simulink model "rp_spectrometer"  (R2021a)
settings: Solver=FixedStepDiscrete  StartTime=0.0  StopTime=10000  RelTol=1e-3
libraries: xbsIndex_r4 x666, casper_library_misc x8, xps_library x3
(part 1 of 11)
settings Model: Creator=hpw1  LastModifiedBy=mcb
settings SolverCC: AlgebraicLoopSolver=TrustRegion
settings DataIOCC: ReturnWorkspaceOutputs=off
settings OptimizationCC: DefaultParameterBehavior=Inlined
settings DebuggingCC: SFMachineParentedDataDiag=warning  ArithmeticOperatorsInVariantConditions=warning
settings SFSimCC: SimUseLocalCustomCode=off  CustomCodeUndefinedFunction=UseInterfaceOnly
settings RTWCC: RTWUseLocalCustomCode=off

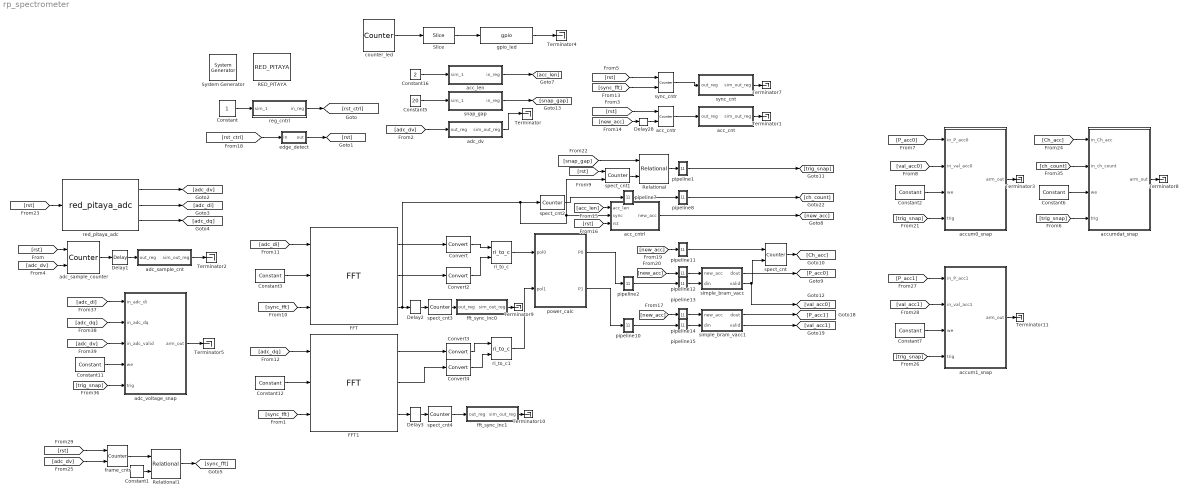
== system rp_spectrometer ==
  " System Generator" : xbsIndex_r4/ System Generator  Tag=genX  xilinxfamily=zynq  part=xc7z010  speed=-1  package=clg400  synthesis_tool=XST  clock_wrapper=Clock Enables  directory=/home/mcb/git/casper/tmp/tutorials_devel/red_pitaya/tut_spec/tut_spec/sysgen  proj_type=Vivado  Synth_file=Vivado Synthesis Defaults  Impl_file=Vivado Implementation Defaults  testbench=off  simulink_period=1  sysclk_period=8  dcm_input_clock_period=10  incr_netlist=off  trim_vbits=Everywhere in SubSystem  dbl_ovrd=According to Block Masks  core_generation=According to Block Masks  run_coregen=off  deprecated_control=off  eval_field=0  block_type=sysgen
  Constant : Constant
  Constant1 : xbsIndex_r4/Constant  const=2^8-1  gui_display_data_type=Fixed-point  arith_type=Unsigned  n_bits=8  bin_pt=0  preci_type=Single  exp_width=8  frac_width=24  explicit_period=off  period=1  equ=P=C  opselect=C  inp2=PCIN>>17  opr=+  inp1=P  carry=CIN  dbl_ovrd=off  block_type=constant
  Constant{2,6..7,11} (4 alike) : xbsIndex_r4/Constant  const=1.0  gui_display_data_type=Boolean  arith_type=Boolean  n_bits=16  bin_pt=14  preci_type=Single  exp_width=8  frac_width=24  explicit_period=on  period=1  equ=P=C  opselect=C  inp2=PCIN>>17  opr=+  inp1=P  carry=CIN  dbl_ovrd=off  block_type=constant
  Constant12 : xbsIndex_r4/Constant  const=0  gui_display_data_type=Fixed-point  arith_type=Signed (2's comp)  n_bits=14  bin_pt=0  preci_type=Single  exp_width=8  frac_width=24  explicit_period=on  period=1  equ=P=C  opselect=C  inp2=PCIN>>17  opr=+  inp1=P  carry=CIN  dbl_ovrd=off  block_type=constant
  Constant16 : Constant  Value=2
  Constant3 : xbsIndex_r4/Constant  const=0  gui_display_data_type=Fixed-point  arith_type=Signed (2's comp)  n_bits=14  bin_pt=0  preci_type=Single  exp_width=8  frac_width=24  explicit_period=on  period=1  equ=P=C  opselect=C  inp2=PCIN>>17  opr=+  inp1=P  carry=CIN  dbl_ovrd=off  block_type=constant
  Constant5 : Constant  Value=20
  Convert{,2..4} (4 alike) : xbsIndex_r4/Convert  gui_display_data_type=Fixed-point  arith_type="Signed  (2's comp)"  n_bits=15  bin_pt=0  float_type=Single  exp_bits=8  fraction_bits=24  quantization=Truncate  overflow=Wrap  en=off  latency=1  pipeline=off  dbl_ovrd=off  block_type=convert
  Delay1 : xbsIndex_r4/Delay  rst=off  infoeditControl=Selection of Reset will increase slice count due to use of real FFs and instead of SRLs  en=off  latency=1  reg_retiming=off  dbl_ovrd=off  block_type=delay
  Delay2 : xbsIndex_r4/Delay  rst=off  infoeditControl=Selection of Reset will increase slice count due to use of real FFs and instead of SRLs  en=off  latency=1  reg_retiming=off  dbl_ovrd=off  block_type=delay
  Delay28 : xbsIndex_r4/Delay  rst=off  infoeditControl=Selection of Reset will increase slice count due to use of real FFs and instead of SRLs  en=off  latency=1  reg_retiming=on  dbl_ovrd=off  block_type=delay
  Delay3 : xbsIndex_r4/Delay  rst=off  infoeditControl=Selection of Reset will increase slice count due to use of real FFs and instead of SRLs  en=off  latency=1  reg_retiming=off  dbl_ovrd=off  block_type=delay
  FFT : xbsIndex_r4/FFT  infoeditControl=Hardware notes: This block implements a burst IO radix-2 architecture if the <b><i>Optimize for</i></b> parameter is selected as <b><i>Resources</i></b>, and the input sample period is 8 times slower than the system sample period; otherwise a pipeline streaming architecture will be used.  transform_length=256  scale_result_by_fft_length=off  bit_reversed_order=on  optimizegoal=Performance  start_frame=on  simulation_type=fast_sim  simulation_model=sysgen:ForwardFFT_Macro  latency=1  block_type=xfft_forward
  FFT1 : xbsIndex_r4/FFT  infoeditControl=Hardware notes: This block implements a burst IO radix-2 architecture if the <b><i>Optimize for</i></b> parameter is selected as <b><i>Resources</i></b>, and the input sample period is 8 times slower than the system sample period; otherwise a pipeline streaming architecture will be used.  transform_length=256  scale_result_by_fft_length=off  bit_reversed_order=on  optimizegoal=Performance  start_frame=on  simulation_type=fast_sim  simulation_model=sysgen:ForwardFFT_Macro  latency=1  block_type=xfft_forward
  RED_PITAYA : xps_library/Platforms/RED_PITAYA  Tag=xps:xsg  hw_sys=RED_PITAYA_14:xc7z010  clk_src=sys_clk  clk_rate=125  sample_period=1  synthesis_tool=XST
      settings: SourceProductName=CASPER XPS Blockset
  Relational : xbsIndex_r4/Relational  mode=a=b  op_type=Bool  en=off  latency=0  dbl_ovrd=off  block_type=relational
  Relational1 : xbsIndex_r4/Relational  mode=a=b  op_type=Bool  en=off  latency=0  dbl_ovrd=off  block_type=relational
  Slice : xbsIndex_r4/Slice  nbits=1  boolean_output=off  mode=Upper Bit Location + Width  bit1=0  base1=MSB of Input  bit0=0  base0=LSB of Input  dbl_ovrd=off  block_type=slice
  Terminator{,1..5,7..11} (11 alike) : Terminator
  acc_cnt : Subsystem  Tag=xps:sw_reg  AncestorBlock=xps_library/Memory/software_register  mask(swreg){io_dir=To Processor, io_delay=0, init_val=0, sample_period=1, names=reg, bitwidths=32, bin_pts=0, arith_types=0, sim_port=on, show_format=off}
      mask prompts: io_dir "I/O direction"; io_delay "I/O delay"; init_val "Initial Value"; sample_period "Sample period"; names "Bitfield names [msb...lsb]"; bitwidths "Bitfield widths"; bin_pts "Bitfield binary pts"; arith_types "Bitfield types, ufix=0, fix=1, bool=2"; sim_port "Provide sim input/output?"; show_format "Print format string?"
      mask help: A 32-bit software-accessible register. Can be divided into bitfields of varying widths and types using the fields in the block mask.
      mask init:
      | swreg_init(gcb)
      settings: AttributesFormatString=1output
      mask TypeOptions io_dir: To Processor | From Processor
      mask Callback io_dir:
      | mask_enables = get_param(gcb, 'MaskEnables');
      | mask_names = get_param(gcb, 'MaskNames');
      | if strcmp(get_param(gcb, 'io_dir'), 'To Processor'),
      |     mask_enables{ismember(mask_names, 'sample_period')} = 'off';
      | else
      |     mask_enables{ismember(mask_names, 'sample_period')} = 'on';
      | end
      | set_param(gcb, 'MaskEnables', mask_enables);
      mask DialogControl ParameterTabVar0 Prompt: Setup
  acc_cntr : xbsIndex_r4/Counter  cnt_type=Free Running  cnt_to=Inf  operation=Up  start_count=0  cnt_by_val=1  arith_type=Unsigned  n_bits=32  bin_pt=0  load_pin=off  rst=on  en=on  explicit_period=on  period=1  use_behavioral_HDL=off  implementation=Fabric  use_rpm=off  dbl_ovrd=off  block_type=counter
  acc_cntrl : Subsystem  mask{chan_bits=8}
      mask prompts: chan_bits "Number of Channels (2^?)"
  acc_len : Subsystem  Tag=xps:sw_reg  AncestorBlock=xps_library/Memory/software_register  mask(swreg){io_dir=From Processor, io_delay=0, init_val=2, sample_period=1, names=reg, bitwidths=32, bin_pts=0, arith_types=0, sim_port=on, show_format=off}
      mask prompts: io_dir "I/O direction"; io_delay "I/O delay"; init_val "Initial Value"; sample_period "Sample period"; names "Bitfield names [msb...lsb]"; bitwidths "Bitfield widths"; bin_pts "Bitfield binary pts"; arith_types "Bitfield types, ufix=0, fix=1, bool=2"; sim_port "Provide sim input/output?"; show_format "Print format string?"
      mask help: A 32-bit software-accessible register. Can be divided into bitfields of varying widths and types using the fields in the block mask.
      mask init:
      | swreg_init(gcb)
      settings: AttributesFormatString=1input
      mask TypeOptions io_dir: To Processor | From Processor
      mask Callback io_dir:
      | mask_enables = get_param(gcb, 'MaskEnables');
      | mask_names = get_param(gcb, 'MaskNames');
      | if strcmp(get_param(gcb, 'io_dir'), 'To Processor'),
      |     mask_enables{ismember(mask_names, 'sample_period')} = 'off';
      | else
      |     mask_enables{ismember(mask_names, 'sample_period')} = 'on';
      | end
      | set_param(gcb, 'MaskEnables', mask_enables);
      mask DialogControl ParameterTabVar0 Prompt: Setup
  accum0_snap : Subsystem  Tag=casper:bitsnap  AncestorBlock=casper_library_scopes/bitfield_snapshot  mask(bitsnap){io_names=[P_acc0 val_acc0], io_widths=[31 1], io_bps=0, io_types=[0 2], show_format=on, snap_storage=bram, snap_dram_dimm=2, snap_dram_clock=250, snap_nsamples=12, snap_data_width=32, snap_offset=off, snap_circap=off, snap_value=off, snap_ext_arm=off, snap_ext_circ=off, snap_provide_outputs=on, snap_use_dsp48=on, snap_delay=0, extra_names=[c d], extra_widths=[30 2], extra_bps=[0 0], extra_types=[0 0]}
      mask prompts: io_names "Names [msb...lsb]"; io_widths "Bitwidths [msb...lsb]"; io_bps "Binary pts [msb...lsb]"; io_types "Data types [msb...lsb], ufix=0, fix=1, bool=2"; show_format "Print format string?"; snap_storage "Storage medium"; snap_dram_dimm "DRAM dimm"; snap_dram_clock "DRAM clock rate"; snap_nsamples "Number of Samples (2^?)"; snap_data_width "Data width"; snap_offset "Start delay support"; snap_circap "Circular capture support"; snap_value "Extra value capture support"; snap_ext_arm "External arm support"; snap_ext_circ "External circular capture support"; snap_provide_outputs "Provide outputs"; snap_use_dsp48 "Use DSP48s to implement counters"; snap_delay "Pre-snapshot delay"; extra_names "Names [msb...lsb]"; extra_widths "Widths [msb...lsb]"; extra_bps "Binary pts [msb...lsb]"; extra_types "Data types [msb...lsb], ufix=0, fix=1, bool=2"
      mask help:
      | A wrapped snapshot block. Allows specification of inputs to a snapblock word so the toolflow can automatically set up the scope.
      | See documentation for snapshot for explanation of parameters.
      mask init:
      | bitsnap_init(gcb);
      settings: AttributesFormatString=|
      | snap(2):uf31.0,b = 32 bits\n32 wide, 4096 deep
      | debugID: 97412755
      mask TypeOptions snap_storage: bram | dram
      mask Callback snap_storage: bitsnap_callback();
      mask TypeOptions snap_dram_dimm: 1 | 2 | 3 | 4
      mask TypeOptions snap_dram_clock: 200 | 250 | 266 | 300 | 333
      mask TypeOptions snap_data_width: 8 | 16 | 32 | 64 | 128
      mask Callback snap_value: bitsnap_callback();
      mask Callback snap_ext_arm: bitsnap_callback();
      mask Callback snap_ext_circ: bitsnap_callback();
      mask Callback snap_provide_outputs: bitsnap_callback();
      mask DialogControl ParameterTabVar0 Prompt: Inputs
      mask DialogControl ParameterTabVar01 Prompt: Snapshot
      mask DialogControl ParameterTabVar012 Prompt: Extra Value
  accum1_snap : Subsystem  Tag=casper:bitsnap  AncestorBlock=casper_library_scopes/bitfield_snapshot  mask(bitsnap){io_names=[P_acc1 val_acc1], io_widths=[31 1], io_bps=0, io_types=[0 2], show_format=on, snap_storage=bram, snap_dram_dimm=2, snap_dram_clock=250, snap_nsamples=12, snap_data_width=32, snap_offset=off, snap_circap=off, snap_value=off, snap_ext_arm=off, snap_ext_circ=off, snap_provide_outputs=on, snap_use_dsp48=on, snap_delay=0, extra_names=[c d], extra_widths=[30 2], extra_bps=[0 0], extra_types=[0 0]}
      mask prompts: io_names "Names [msb...lsb]"; io_widths "Bitwidths [msb...lsb]"; io_bps "Binary pts [msb...lsb]"; io_types "Data types [msb...lsb], ufix=0, fix=1, bool=2"; show_format "Print format string?"; snap_storage "Storage medium"; snap_dram_dimm "DRAM dimm"; snap_dram_clock "DRAM clock rate"; snap_nsamples "Number of Samples (2^?)"; snap_data_width "Data width"; snap_offset "Start delay support"; snap_circap "Circular capture support"; snap_value "Extra value capture support"; snap_ext_arm "External arm support"; snap_ext_circ "External circular capture support"; snap_provide_outputs "Provide outputs"; snap_use_dsp48 "Use DSP48s to implement counters"; snap_delay "Pre-snapshot delay"; extra_names "Names [msb...lsb]"; extra_widths "Widths [msb...lsb]"; extra_bps "Binary pts [msb...lsb]"; extra_types "Data types [msb...lsb], ufix=0, fix=1, bool=2"
      mask help:
      | A wrapped snapshot block. Allows specification of inputs to a snapblock word so the toolflow can automatically set up the scope.
      | See documentation for snapshot for explanation of parameters.
      mask init:
      | bitsnap_init(gcb);
      settings: AttributesFormatString=|
      | snap(2):uf31.0,b = 32 bits\n32 wide, 4096 deep
      | debugID: 34788756
      mask TypeOptions snap_storage: bram | dram
      mask Callback snap_storage: bitsnap_callback();
      mask TypeOptions snap_dram_dimm: 1 | 2 | 3 | 4
      mask TypeOptions snap_dram_clock: 200 | 250 | 266 | 300 | 333
      mask TypeOptions snap_data_width: 8 | 16 | 32 | 64 | 128
      mask Callback snap_value: bitsnap_callback();
      mask Callback snap_ext_arm: bitsnap_callback();
      mask Callback snap_ext_circ: bitsnap_callback();
      mask Callback snap_provide_outputs: bitsnap_callback();
      mask DialogControl ParameterTabVar0 Prompt: Inputs
      mask DialogControl ParameterTabVar01 Prompt: Snapshot
      mask DialogControl ParameterTabVar012 Prompt: Extra Value
  accumdat_snap : Subsystem  Tag=casper:bitsnap  AncestorBlock=casper_library_scopes/bitfield_snapshot  mask(bitsnap){io_names=[Ch_acc ch_count], io_widths=[11 8], io_bps=0, io_types=[0 0], show_format=on, snap_storage=bram, snap_dram_dimm=2, snap_dram_clock=250, snap_nsamples=12, snap_data_width=32, snap_offset=off, snap_circap=off, snap_value=off, snap_ext_arm=off, snap_ext_circ=off, snap_provide_outputs=on, snap_use_dsp48=on, snap_delay=0, extra_names=[c d], extra_widths=[30 2], extra_bps=[0 0], extra_types=[0 0]}
      mask prompts: io_names "Names [msb...lsb]"; io_widths "Bitwidths [msb...lsb]"; io_bps "Binary pts [msb...lsb]"; io_types "Data types [msb...lsb], ufix=0, fix=1, bool=2"; show_format "Print format string?"; snap_storage "Storage medium"; snap_dram_dimm "DRAM dimm"; snap_dram_clock "DRAM clock rate"; snap_nsamples "Number of Samples (2^?)"; snap_data_width "Data width"; snap_offset "Start delay support"; snap_circap "Circular capture support"; snap_value "Extra value capture support"; snap_ext_arm "External arm support"; snap_ext_circ "External circular capture support"; snap_provide_outputs "Provide outputs"; snap_use_dsp48 "Use DSP48s to implement counters"; snap_delay "Pre-snapshot delay"; extra_names "Names [msb...lsb]"; extra_widths "Widths [msb...lsb]"; extra_bps "Binary pts [msb...lsb]"; extra_types "Data types [msb...lsb], ufix=0, fix=1, bool=2"
      mask help:
      | A wrapped snapshot block. Allows specification of inputs to a snapblock word so the toolflow can automatically set up the scope.
      | See documentation for snapshot for explanation of parameters.
      mask init:
      | bitsnap_init(gcb);
      settings: AttributesFormatString=|
      | snap(2):uf11.0,uf8.0 = 19 bits\n32 wide, 4096 deep
      | debugID: 7196602
      mask TypeOptions snap_storage: bram | dram
      mask Callback snap_storage: bitsnap_callback();
      mask TypeOptions snap_dram_dimm: 1 | 2 | 3 | 4
      mask TypeOptions snap_dram_clock: 200 | 250 | 266 | 300 | 333
      mask TypeOptions snap_data_width: 8 | 16 | 32 | 64 | 128
      mask Callback snap_value: bitsnap_callback();
      mask Callback snap_ext_arm: bitsnap_callback();
      mask Callback snap_ext_circ: bitsnap_callback();
      mask Callback snap_provide_outputs: bitsnap_callback();
      mask DialogControl ParameterTabVar0 Prompt: Inputs
      mask DialogControl ParameterTabVar01 Prompt: Snapshot
      mask DialogControl ParameterTabVar012 Prompt: Extra Value
  adc_dv : Subsystem  Tag=xps:sw_reg  AncestorBlock=xps_library/Memory/software_register  mask(swreg){io_dir=To Processor, io_delay=0, init_val=0, sample_period=1, names=reg, bitwidths=1, bin_pts=0, arith_types=2, sim_port=on, show_format=on}
      mask prompts: io_dir "I/O direction"; io_delay "I/O delay"; init_val "Initial Value"; sample_period "Sample period"; names "Bitfield names [msb...lsb]"; bitwidths "Bitfield widths"; bin_pts "Bitfield binary pts"; arith_types "Bitfield types, ufix=0, fix=1, bool=2"; sim_port "Provide sim input/output?"; show_format "Print format string?"
      mask help: A 32-bit software-accessible register. Can be divided into bitfields of varying widths and types using the fields in the block mask.
      mask init:
      | swreg_init(gcb)
      settings: AttributesFormatString=1output:b = 1 bits
      mask TypeOptions io_dir: To Processor | From Processor
      mask Callback io_dir:
      | mask_enables = get_param(gcb, 'MaskEnables');
      | mask_names = get_param(gcb, 'MaskNames');
      | if strcmp(get_param(gcb, 'io_dir'), 'To Processor'),
      |     mask_enables{ismember(mask_names, 'sample_period')} = 'off';
      | else
      |     mask_enables{ismember(mask_names, 'sample_period')} = 'on';
      | end
      | set_param(gcb, 'MaskEnables', mask_enables);
      mask DialogControl ParameterTabVar0 Prompt: Setup
  adc_sample_cnt : Subsystem  Tag=xps:sw_reg  AncestorBlock=xps_library/Memory/software_register  mask(swreg){io_dir=To Processor, io_delay=0, init_val=0, sample_period=1, names=reg, bitwidths=32, bin_pts=0, arith_types=0, sim_port=on, show_format=on}
      mask prompts: io_dir "I/O direction"; io_delay "I/O delay"; init_val "Initial Value"; sample_period "Sample period"; names "Bitfield names [msb...lsb]"; bitwidths "Bitfield widths"; bin_pts "Bitfield binary pts"; arith_types "Bitfield types, ufix=0, fix=1, bool=2"; sim_port "Provide sim input/output?"; show_format "Print format string?"
      mask help: A 32-bit software-accessible register. Can be divided into bitfields of varying widths and types using the fields in the block mask.
      mask init:
      | swreg_init(gcb)
      settings: AttributesFormatString=1output:uf32.0 = 32 bits
      mask TypeOptions io_dir: To Processor | From Processor
      mask Callback io_dir:
      | mask_enables = get_param(gcb, 'MaskEnables');
      | mask_names = get_param(gcb, 'MaskNames');
      | if strcmp(get_param(gcb, 'io_dir'), 'To Processor'),
      |     mask_enables{ismember(mask_names, 'sample_period')} = 'off';
      | else
      |     mask_enables{ismember(mask_names, 'sample_period')} = 'on';
      | end
      | set_param(gcb, 'MaskEnables', mask_enables);
      mask DialogControl ParameterTabVar0 Prompt: Setup
  adc_sample_counter : xbsIndex_r4/Counter  cnt_type=Free Running  cnt_to=Inf  operation=Up  start_count=0  cnt_by_val=1  arith_type=Unsigned  n_bits=32  bin_pt=0  load_pin=off  rst=on  en=on  explicit_period=on  period=1  use_behavioral_HDL=off  implementation=Fabric  dbl_ovrd=off  block_type=counter
  adc_voltage_snap : Subsystem  Tag=casper:bitsnap  AncestorBlock=casper_library_scopes/bitfield_snapshot  mask(bitsnap){io_names=[adc_di adc_dq adc_valid], io_widths=[14 14 1], io_bps=0, io_types=[1 1 2], show_format=on, snap_storage=bram, snap_dram_dimm=2, snap_dram_clock=250, snap_nsamples=12, snap_data_width=32, snap_offset=off, snap_circap=off, snap_value=off, snap_ext_arm=off, snap_ext_circ=off, snap_provide_outputs=on, snap_use_dsp48=on, snap_delay=0, extra_names=[c d], extra_widths=[30 2], extra_bps=[0 0], extra_types=[0 0]}
      mask prompts: io_names "Names [msb...lsb]"; io_widths "Bitwidths [msb...lsb]"; io_bps "Binary pts [msb...lsb]"; io_types "Data types [msb...lsb], ufix=0, fix=1, bool=2"; show_format "Print format string?"; snap_storage "Storage medium"; snap_dram_dimm "DRAM dimm"; snap_dram_clock "DRAM clock rate"; snap_nsamples "Number of Samples (2^?)"; snap_data_width "Data width"; snap_offset "Start delay support"; snap_circap "Circular capture support"; snap_value "Extra value capture support"; snap_ext_arm "External arm support"; snap_ext_circ "External circular capture support"; snap_provide_outputs "Provide outputs"; snap_use_dsp48 "Use DSP48s to implement counters"; snap_delay "Pre-snapshot delay"; extra_names "Names [msb...lsb]"; extra_widths "Widths [msb...lsb]"; extra_bps "Binary pts [msb...lsb]"; extra_types "Data types [msb...lsb], ufix=0, fix=1, bool=2"
      mask help:
      | A wrapped snapshot block. Allows specification of inputs to a snapblock word so the toolflow can automatically set up the scope.
      | See documentation for snapshot for explanation of parameters.
      mask init:
      | bitsnap_init(gcb);
      settings: AttributesFormatString=|
      | snap(3):f14.0,f14.0,b = 29 bits\n32 wide, 4096 deep
      | debugID: 53243759
      mask TypeOptions snap_storage: bram | dram
      mask Callback snap_storage: bitsnap_callback();
      mask TypeOptions snap_dram_dimm: 1 | 2 | 3 | 4
      mask TypeOptions snap_dram_clock: 200 | 250 | 266 | 300 | 333
      mask TypeOptions snap_data_width: 8 | 16 | 32 | 64 | 128
      mask Callback snap_value: bitsnap_callback();
      mask Callback snap_ext_arm: bitsnap_callback();
      mask Callback snap_ext_circ: bitsnap_callback();
      mask Callback snap_provide_outputs: bitsnap_callback();
      mask DialogControl ParameterTabVar0 Prompt: Inputs
      mask DialogControl ParameterTabVar01 Prompt: Snapshot
      mask DialogControl ParameterTabVar012 Prompt: Extra Value
  counter_led : xbsIndex_r4/Counter  cnt_type=Free Running  cnt_to=Inf  operation=Up  start_count=0  cnt_by_val=1  arith_type=Unsigned  n_bits=27  bin_pt=0  load_pin=off  rst=off  en=off  explicit_period=on  period=1  use_behavioral_HDL=off  implementation=Fabric  dbl_ovrd=off  block_type=counter
  edge_detect : Subsystem  AncestorBlock=casper_library_misc/edge_detect  mask(edge_detect){edge=Rising, polarity=Active High, x_in=[0 0.08 0.08 0.16 0.16 0.24 0.24 0.32 0.32 0.4], y_in=[-1 -1  1  1  1  1  1  1  1  1], x_out=[0.6 0.68 0.68 0.76 0.76 0.84 0.84 0.92 0.92 1], y_out=[-1 -1  1  1 -1 -1 -1 -1 -1 -1]}
      mask prompts: edge "Edge Type"; polarity "Output Polarity"; x_in "Input X Positions"; y_in "Input Y Positions"; x_out "Output X Positions"; y_out "Output Y Positions"
      mask help: Output is active for one-cycle after each edge of the specified type (i.e. rising, falling or both).
      mask init:
      | edge_detect_init(gcb,...
      |     'edge',edge,...
      |     'polarity',polarity,...
      |     'x_in',x_in,...
      |     'x_out',x_out,...
      |     'y_in',y_in,...
      |     'y_out',y_out);
      | 
      | x_in_num=str2num(getfield(getfield(get_param(gcb,'UserData'),'parameters'),'x_in'));
      | x_out_num=str2num(getfield(getfield(get_param(gcb,'UserData'),'parameters'),'x_out'));
      | y_in_num=str2num(getfield(getfield(get_param(gcb,'UserData'),'parameters'),'y_in'));
      | y_out_num=str2num(getfield(getfield(get_param(gcb,'UserData'),'parameters'),'y_out'));
      settings: AttributesFormatString=|
      | rising edges
      | active high
      mask Help: Output is active for one-cycle after each edge of the specified type (i.e. rising, falling, or both).  Latency is zero.
      mask TypeOptions edge: Rising | Falling | Both
      mask TypeOptions polarity: Active High | Active Low
      mask Display:
      | plot(x_in_num,0.5+y_in_num*0.2);
      | plot(x_out_num,0.5+y_out_num*0.2);
  fft_sync_inc0 : Subsystem  Tag=xps:sw_reg  AncestorBlock=xps_library/Memory/software_register  mask(swreg){io_dir=To Processor, io_delay=0, init_val=0, sample_period=1, names=reg, bitwidths=8, bin_pts=0, arith_types=0, sim_port=on, show_format=on}
      mask prompts: io_dir "I/O direction"; io_delay "I/O delay"; init_val "Initial Value"; sample_period "Sample period"; names "Bitfield names [msb...lsb]"; bitwidths "Bitfield widths"; bin_pts "Bitfield binary pts"; arith_types "Bitfield types, ufix=0, fix=1, bool=2"; sim_port "Provide sim input/output?"; show_format "Print format string?"
      mask help: A 32-bit software-accessible register. Can be divided into bitfields of varying widths and types using the fields in the block mask.
      mask init:
      | swreg_init(gcb)
      settings: AttributesFormatString=1output:uf8.0 = 8 bits
      mask TypeOptions io_dir: To Processor | From Processor
      mask Callback io_dir:
      | mask_enables = get_param(gcb, 'MaskEnables');
      | mask_names = get_param(gcb, 'MaskNames');
      | if strcmp(get_param(gcb, 'io_dir'), 'To Processor'),
      |     mask_enables{ismember(mask_names, 'sample_period')} = 'off';
      | else
      |     mask_enables{ismember(mask_names, 'sample_period')} = 'on';
      | end
      | set_param(gcb, 'MaskEnables', mask_enables);
      mask DialogControl ParameterTabVar0 Prompt: Setup
  fft_sync_inc1 : Subsystem  Tag=xps:sw_reg  AncestorBlock=xps_library/Memory/software_register  mask(swreg){io_dir=To Processor, io_delay=0, init_val=0, sample_period=1, names=reg, bitwidths=8, bin_pts=0, arith_types=0, sim_port=on, show_format=on}
      mask prompts: io_dir "I/O direction"; io_delay "I/O delay"; init_val "Initial Value"; sample_period "Sample period"; names "Bitfield names [msb...lsb]"; bitwidths "Bitfield widths"; bin_pts "Bitfield binary pts"; arith_types "Bitfield types, ufix=0, fix=1, bool=2"; sim_port "Provide sim input/output?"; show_format "Print format string?"
      mask help: A 32-bit software-accessible register. Can be divided into bitfields of varying widths and types using the fields in the block mask.
      mask init:
      | swreg_init(gcb)
      settings: AttributesFormatString=1output:uf8.0 = 8 bits
      mask TypeOptions io_dir: To Processor | From Processor
      mask Callback io_dir:
      | mask_enables = get_param(gcb, 'MaskEnables');
      | mask_names = get_param(gcb, 'MaskNames');
      | if strcmp(get_param(gcb, 'io_dir'), 'To Processor'),
      |     mask_enables{ismember(mask_names, 'sample_period')} = 'off';
      | else
      |     mask_enables{ismember(mask_names, 'sample_period')} = 'on';
      | end
      | set_param(gcb, 'MaskEnables', mask_enables);
      mask DialogControl ParameterTabVar0 Prompt: Setup
  frame_cntr : xbsIndex_r4/Counter  cnt_type=Free Running  cnt_to=Inf  operation=Up  start_count=0  cnt_by_val=1  arith_type=Unsigned  n_bits=8  bin_pt=0  load_pin=off  rst=on  en=on  explicit_period=on  period=1  use_behavioral_HDL=off  implementation=Fabric  dbl_ovrd=off  block_type=counter
  gpio_led : xps_library/IO/gpio  Tag=xps:gpio  io_group_params_forwarded=on  io_group=ROACH:led  io_group_real=led  io_group_custom=0  io_dir=out  arith_type=Boolean  bitwidth=1  bin_pt=0  bit_index=0  sample_period=1  use_single_ended=off  use_ddr=off  reg_iob=on  reg_clk_phase=0  termination=None  use_iodelay=off
      settings: SourceProductName=CASPER XPS Blockset
  pipeline1 : Subsystem  AncestorBlock=casper_library_delays/pipeline  mask(pipeline){csp_latency=1}
      mask prompts: csp_latency "Latency"
      mask help:
      | An explicitly laid-out delay line to avoid mapping to SRL16s
      | for use in pipelining to help achieve timing closure.
      mask init:
      | pipeline_init(gcb,'latency',csp_latency);
      settings: AttributesFormatString=Latency = %<latency>
      mask Display:
      | port_label('input', 1, 'd');
      | port_label('output', 1, 'q');
      | disp(['Z^-', num2str(csp_latency)]);
  pipeline10 : Subsystem  AncestorBlock=casper_library_delays/pipeline  mask(pipeline){csp_latency=1}
      mask prompts: csp_latency "Latency"
      mask help:
      | An explicitly laid-out delay line to avoid mapping to SRL16s
      | for use in pipelining to help achieve timing closure.
      mask init:
      | pipeline_init(gcb,'latency',csp_latency);
      settings: AttributesFormatString=Latency = %<latency>
      mask Display:
      | port_label('input', 1, 'd');
      | port_label('output', 1, 'q');
      | disp(['Z^-', num2str(csp_latency)]);
  pipeline11 : Subsystem  AncestorBlock=casper_library_delays/pipeline  mask(pipeline){csp_latency=1}
      mask prompts: csp_latency "Latency"
      mask help:
      | An explicitly laid-out delay line to avoid mapping to SRL16s
      | for use in pipelining to help achieve timing closure.
      mask init:
      | pipeline_init(gcb,'latency',csp_latency);
      settings: AttributesFormatString=Latency = %<latency>
      mask Display:
      | port_label('input', 1, 'd');
      | port_label('output', 1, 'q');
      | disp(['Z^-', num2str(csp_latency)]);
  pipeline12 : Subsystem  AncestorBlock=casper_library_delays/pipeline  mask(pipeline){csp_latency=1}
      mask prompts: csp_latency "Latency"
      mask help:
      | An explicitly laid-out delay line to avoid mapping to SRL16s
      | for use in pipelining to help achieve timing closure.
      mask init:
      | pipeline_init(gcb,'latency',csp_latency);
      settings: AttributesFormatString=Latency = %<latency>
      mask Display:
      | port_label('input', 1, 'd');
      | port_label('output', 1, 'q');
      | disp(['Z^-', num2str(csp_latency)]);
  pipeline13 : Subsystem  AncestorBlock=casper_library_delays/pipeline  mask(pipeline){csp_latency=1}
      mask prompts: csp_latency "Latency"
      mask help:
      | An explicitly laid-out delay line to avoid mapping to SRL16s
      | for use in pipelining to help achieve timing closure.
      mask init:
      | pipeline_init(gcb,'latency',csp_latency);
      settings: AttributesFormatString=Latency = %<latency>
      mask Display:
      | port_label('input', 1, 'd');
      | port_label('output', 1, 'q');
      | disp(['Z^-', num2str(csp_latency)]);
  pipeline14 : Subsystem  AncestorBlock=casper_library_delays/pipeline  mask(pipeline){csp_latency=1}
      mask prompts: csp_latency "Latency"
      mask help:
      | An explicitly laid-out delay line to avoid mapping to SRL16s
      | for use in pipelining to help achieve timing closure.
      mask init:
      | pipeline_init(gcb,'latency',csp_latency);
      settings: AttributesFormatString=Latency = %<latency>
      mask Display:
      | port_label('input', 1, 'd');
      | port_label('output', 1, 'q');
      | disp(['Z^-', num2str(csp_latency)]);
  pipeline15 : Subsystem  AncestorBlock=casper_library_delays/pipeline  mask(pipeline){csp_latency=1}
      mask prompts: csp_latency "Latency"
      mask help:
      | An explicitly laid-out delay line to avoid mapping to SRL16s
      | for use in pipelining to help achieve timing closure.
      mask init:
      | pipeline_init(gcb,'latency',csp_latency);
      settings: AttributesFormatString=Latency = %<latency>
      mask Display:
      | port_label('input', 1, 'd');
      | port_label('output', 1, 'q');
      | disp(['Z^-', num2str(csp_latency)]);
  pipeline2 : Subsystem  AncestorBlock=casper_library_delays/pipeline  mask(pipeline){csp_latency=1}
      mask prompts: csp_latency "Latency"
      mask help:
      | An explicitly laid-out delay line to avoid mapping to SRL16s
      | for use in pipelining to help achieve timing closure.
      mask init:
      | pipeline_init(gcb,'latency',csp_latency);
      settings: AttributesFormatString=Latency = %<latency>
      mask Display:
      | port_label('input', 1, 'd');
      | port_label('output', 1, 'q');
      | disp(['Z^-', num2str(csp_latency)]);
  pipeline7 : Subsystem  AncestorBlock=casper_library_delays/pipeline  mask(pipeline){csp_latency=1}
      mask prompts: csp_latency "Latency"
      mask help:
      | An explicitly laid-out delay line to avoid mapping to SRL16s
      | for use in pipelining to help achieve timing closure.
      mask init:
      | pipeline_init(gcb,'latency',csp_latency);
      settings: AttributesFormatString=Latency = %<latency>
      mask Display:
      | port_label('input', 1, 'd');
      | port_label('output', 1, 'q');
      | disp(['Z^-', num2str(csp_latency)]);
  pipeline8 : Subsystem  AncestorBlock=casper_library_delays/pipeline  mask(pipeline){csp_latency=1}
      mask prompts: csp_latency "Latency"
      mask help:
      | An explicitly laid-out delay line to avoid mapping to SRL16s
      | for use in pipelining to help achieve timing closure.
      mask init:
      | pipeline_init(gcb,'latency',csp_latency);
      settings: AttributesFormatString=Latency = %<latency>
      mask Display:
      | port_label('input', 1, 'd');
      | port_label('output', 1, 'q');
      | disp(['Z^-', num2str(csp_latency)]);
  power_calc : Subsystem
  red_pitaya_adc : xps_library/ADCs/red_pitaya_adc  Tag=xps:red_pitaya_adc  bits=14
      settings: SourceProductName=CASPER XPS Blockset
  reg_cntrl : Subsystem  Tag=xps:sw_reg  AncestorBlock=xps_library/Memory/software_register  mask(swreg){io_dir=From Processor, io_delay=0, init_val=0, sample_period=1, names=reg, bitwidths=1, bin_pts=0, arith_types=2, sim_port=on, show_format=on}
      mask prompts: io_dir "I/O direction"; io_delay "I/O delay"; init_val "Initial Value"; sample_period "Sample period"; names "Bitfield names [msb...lsb]"; bitwidths "Bitfield widths"; bin_pts "Bitfield binary pts"; arith_types "Bitfield types, ufix=0, fix=1, bool=2"; sim_port "Provide sim input/output?"; show_format "Print format string?"
      mask help: A 32-bit software-accessible register. Can be divided into bitfields of varying widths and types using the fields in the block mask.
      mask init:
      | swreg_init(gcb)
      settings: AttributesFormatString=1input:b = 1 bits
      mask TypeOptions io_dir: To Processor | From Processor
      mask Callback io_dir:
      | mask_enables = get_param(gcb, 'MaskEnables');
      | mask_names = get_param(gcb, 'MaskNames');
      | if strcmp(get_param(gcb, 'io_dir'), 'To Processor'),
      |     mask_enables{ismember(mask_names, 'sample_period')} = 'off';
      | else
      |     mask_enables{ismember(mask_names, 'sample_period')} = 'on';
      | end
      | set_param(gcb, 'MaskEnables', mask_enables);
      mask DialogControl ParameterTabVar0 Prompt: Setup
  ri_to_c : casper_library_misc/ri_to_c
      settings: SourceProductName=CASPER DSP Blockset
  ri_to_c1 : casper_library_misc/ri_to_c
      settings: SourceProductName=CASPER DSP Blockset
  simple_bram_vacc : Subsystem  AncestorBlock=casper_library_accumulators/simple_bram_vacc  mask(simple_bram_vacc){vec_len=256, arith_type=Unsigned, n_bits=31, bin_pt=0}
      mask prompts: vec_len "Vector length:"; arith_type "Output type:"; n_bits "Bit width (output):"; bin_pt "Binary point (output):"
      mask help: This simple vector accumulator is based on a shift register. It outputs its previous accumulated vector after a new_acc pulse is received.
      mask init:
      | simple_bram_vacc_init(gcb, ...
      |     'vec_len', vec_len, ...
      |     'arith_type', arith_type, ...
      |     'n_bits', n_bits, ...
      |     'bin_pt', bin_pt);
      mask TypeOptions arith_type: Signed | Unsigned
  simple_bram_vacc1 : Subsystem  AncestorBlock=casper_library_accumulators/simple_bram_vacc  mask(simple_bram_vacc){vec_len=256, arith_type=Unsigned, n_bits=31, bin_pt=0}
      mask prompts: vec_len "Vector length:"; arith_type "Output type:"; n_bits "Bit width (output):"; bin_pt "Binary point (output):"
      mask help: This simple vector accumulator is based on a shift register. It outputs its previous accumulated vector after a new_acc pulse is received.
      mask init:
      | simple_bram_vacc_init(gcb, ...
      |     'vec_len', vec_len, ...
      |     'arith_type', arith_type, ...
      |     'n_bits', n_bits, ...
      |     'bin_pt', bin_pt);
      mask TypeOptions arith_type: Signed | Unsigned
  snap_gap : Subsystem  Tag=xps:sw_reg  AncestorBlock=xps_library/Memory/software_register  mask(swreg){io_dir=From Processor, io_delay=0, init_val=20, sample_period=1, names=reg, bitwidths=32, bin_pts=0, arith_types=0, sim_port=on, show_format=off}
      mask prompts: io_dir "I/O direction"; io_delay "I/O delay"; init_val "Initial Value"; sample_period "Sample period"; names "Bitfield names [msb...lsb]"; bitwidths "Bitfield widths"; bin_pts "Bitfield binary pts"; arith_types "Bitfield types, ufix=0, fix=1, bool=2"; sim_port "Provide sim input/output?"; show_format "Print format string?"
      mask help: A 32-bit software-accessible register. Can be divided into bitfields of varying widths and types using the fields in the block mask.
      mask init:
      | swreg_init(gcb)
      settings: AttributesFormatString=1input
      mask TypeOptions io_dir: To Processor | From Processor
      mask Callback io_dir:
      | mask_enables = get_param(gcb, 'MaskEnables');
      | mask_names = get_param(gcb, 'MaskNames');
      | if strcmp(get_param(gcb, 'io_dir'), 'To Processor'),
      |     mask_enables{ismember(mask_names, 'sample_period')} = 'off';
      | else
      |     mask_enables{ismember(mask_names, 'sample_period')} = 'on';
      | end
      | set_param(gcb, 'MaskEnables', mask_enables);
      mask DialogControl ParameterTabVar0 Prompt: Setup
  spect_cnt : xbsIndex_r4/Counter  cnt_type=Free Running  cnt_to=Inf  operation=Up  start_count=0  cnt_by_val=1  arith_type=Unsigned  n_bits=10+1  bin_pt=0  load_pin=off  rst=on  en=on  explicit_period=on  period=1  use_behavioral_HDL=off  implementation=Fabric  use_rpm=off  dbl_ovrd=off  block_type=counter
  spect_cnt1 : xbsIndex_r4/Counter  cnt_type=Free Running  cnt_to=Inf  operation=Up  start_count=0  cnt_by_val=1  arith_type=Unsigned  n_bits=10+1  bin_pt=0  load_pin=off  rst=on  en=on  explicit_period=on  period=1  use_behavioral_HDL=off  implementation=Fabric  use_rpm=off  dbl_ovrd=off  block_type=counter
  spect_cnt2 : xbsIndex_r4/Counter  cnt_type=Free Running  cnt_to=Inf  operation=Up  start_count=0  cnt_by_val=1  arith_type=Unsigned  n_bits=8  bin_pt=0  load_pin=off  rst=on  en=off  explicit_period=on  period=1  use_behavioral_HDL=off  implementation=Fabric  use_rpm=off  dbl_ovrd=off  block_type=counter
  spect_cnt3 : xbsIndex_r4/Counter  cnt_type=Free Running  cnt_to=Inf  operation=Up  start_count=0  cnt_by_val=1  arith_type=Unsigned  n_bits=8  bin_pt=0  load_pin=off  rst=off  en=on  explicit_period=on  period=1  use_behavioral_HDL=off  implementation=Fabric  use_rpm=off  dbl_ovrd=off  block_type=counter
  spect_cnt4 : xbsIndex_r4/Counter  cnt_type=Free Running  cnt_to=Inf  operation=Up  start_count=0  cnt_by_val=1  arith_type=Unsigned  n_bits=8  bin_pt=0  load_pin=off  rst=off  en=on  explicit_period=on  period=1  use_behavioral_HDL=off  implementation=Fabric  use_rpm=off  dbl_ovrd=off  block_type=counter
  sync_cnt : Subsystem  Tag=xps:sw_reg  AncestorBlock=xps_library/Memory/software_register  mask(swreg){io_dir=To Processor, io_delay=0, init_val=0, sample_period=1, names=reg, bitwidths=32, bin_pts=0, arith_types=0, sim_port=on, show_format=off}
      mask prompts: io_dir "I/O direction"; io_delay "I/O delay"; init_val "Initial Value"; sample_period "Sample period"; names "Bitfield names [msb...lsb]"; bitwidths "Bitfield widths"; bin_pts "Bitfield binary pts"; arith_types "Bitfield types, ufix=0, fix=1, bool=2"; sim_port "Provide sim input/output?"; show_format "Print format string?"
      mask help: A 32-bit software-accessible register. Can be divided into bitfields of varying widths and types using the fields in the block mask.
      mask init:
      | swreg_init(gcb)
      settings: AttributesFormatString=1output
      mask TypeOptions io_dir: To Processor | From Processor
      mask Callback io_dir:
      | mask_enables = get_param(gcb, 'MaskEnables');
      | mask_names = get_param(gcb, 'MaskNames');
      | if strcmp(get_param(gcb, 'io_dir'), 'To Processor'),
      |     mask_enables{ismember(mask_names, 'sample_period')} = 'off';
      | else
      |     mask_enables{ismember(mask_names, 'sample_period')} = 'on';
      | end
      | set_param(gcb, 'MaskEnables', mask_enables);
      mask DialogControl ParameterTabVar0 Prompt: Setup
  sync_cntr : xbsIndex_r4/Counter  cnt_type=Free Running  cnt_to=Inf  operation=Up  start_count=0  cnt_by_val=1  arith_type=Unsigned  n_bits=32  bin_pt=0  load_pin=off  rst=on  en=on  explicit_period=on  period=1  use_behavioral_HDL=off  implementation=Fabric  use_rpm=off  dbl_ovrd=off  block_type=counter
  wires:
  gpio_led/1 -> Terminator4/1
  counter_led/1 -> Slice/1
  Slice/1 -> gpio_led/1
  [rst_ctrl] -> edge_detect/1(in)
  edge_detect/1(out) -> [rst]
  Constant/1 -> reg_cntrl/1(sim_1)
  [adc_dv] -> adc_dv/1(out_reg)
  adc_sample_cnt/1(sim_out_reg) -> Terminator2/1
  [adc_dv] -> adc_sample_counter/2
  adc_sample_counter/1 -> Delay1/1
  Delay1/1 -> adc_sample_cnt/1(out_reg)
  [rst] -> adc_sample_counter/1
  [sync_fft] -> FFT/3
  Constant16/1 -> acc_len/1(sim_1)
  acc_len/1(in_reg) -> [acc_len]
  sync_cnt/1(sim_out_reg) -> Terminator7/1
  [rst] -> acc_cntr/1
  sync_cntr/1 -> sync_cnt/1(out_reg)
  acc_cntr/1 -> acc_cnt/1(out_reg)
  [new_acc] -> Delay28/1
  Delay28/1 -> acc_cntr/2
  acc_cnt/1(sim_out_reg) -> Terminator1/1
  [rst] -> sync_cntr/1
  [sync_fft] -> sync_cntr/2
  [rst] -> acc_cntrl/3(rst)
  [acc_len] -> acc_cntrl/1(acc_len)
  simple_bram_vacc/2(valid) -> [val_acc0], spect_cnt/2
  pipeline13/1(q) -> simple_bram_vacc/2(din)
  pipeline15/1(q) -> simple_bram_vacc1/2(din)
  power_calc/2(P1) -> pipeline10/1(d)
  [new_acc] -> pipeline11/1(d)
  power_calc/1(P0) -> pipeline2/1(d)
  spect_cnt/1 -> [Ch_acc]
  [new_acc] -> pipeline14/1(d)
  [new_acc] -> pipeline12/1(d)
  pipeline14/1(q) -> simple_bram_vacc1/1(new_acc)
  pipeline10/1(q) -> pipeline15/1(d)
  pipeline12/1(q) -> simple_bram_vacc/1(new_acc)
  pipeline2/1(q) -> pipeline13/1(d)
  simple_bram_vacc/1(dout) -> [P_acc0]
  simple_bram_vacc1/1(dout) -> [P_acc1]
  simple_bram_vacc1/2(valid) -> [val_acc1]
  acc_cntrl/1(new_acc) -> [new_acc]
  accum0_snap/1(arm_out) -> Terminator3/1
  Constant2/1 -> accum0_snap/3(we)
  [rst] -> spect_cnt1/1
  spect_cnt1/1 -> Relational/2
  [snap_gap] -> Relational/1
  Relational/1 -> pipeline1/1(d)
  pipeline1/1(q) -> [trig_snap]
  [trig_snap] -> accum0_snap/4(trig)
  pipeline11/1(q) -> spect_cnt/1
  snap_gap/1(in_reg) -> [snap_gap]
  Constant5/1 -> snap_gap/1(sim_1)
  red_pitaya_adc/2 -> [adc_di]
  red_pitaya_adc/3 -> [adc_dq]
  red_pitaya_adc/1 -> [adc_dv]
  [rst] -> red_pitaya_adc/1
  [P_acc0] -> accum0_snap/1(in_P_acc0)
  [val_acc0] -> accum0_snap/2(in_val_acc0)
  accumdat_snap/1(arm_out) -> Terminator8/1
  Constant6/1 -> accumdat_snap/3(we)
  [trig_snap] -> accumdat_snap/4(trig)
  [Ch_acc] -> accumdat_snap/1(in_Ch_acc)
  accum1_snap/1(arm_out) -> Terminator11/1
  Constant7/1 -> accum1_snap/3(we)
  [trig_snap] -> accum1_snap/4(trig)
  [P_acc1] -> accum1_snap/1(in_P_acc1)
  [val_acc1] -> accum1_snap/2(in_val_acc1)
  adc_dv/1(sim_out_reg) -> Terminator/1
  spect_cnt2/1 -> pipeline7/1(d)
  pipeline7/1(q) -> pipeline8/1(d)
  pipeline8/1(q) -> [ch_count]
  [ch_count] -> accumdat_snap/2(in_ch_count)
  reg_cntrl/1(in_reg) -> [rst_ctrl]
  [adc_di] -> adc_voltage_snap/1(in_adc_di)
  [adc_dq] -> adc_voltage_snap/2(in_adc_dq)
  [trig_snap] -> adc_voltage_snap/5(trig)
  Constant11/1 -> adc_voltage_snap/4(we)
  [adc_dv] -> adc_voltage_snap/3(in_adc_valid)
  spect_cnt3/1 -> fft_sync_inc0/1(out_reg)
  FFT/1 -> Convert/1
  FFT/2 -> Convert2/1
  [adc_di] -> FFT/1
  Constant3/1 -> FFT/2
  Convert/1 -> ri_to_c/1
  Convert2/1 -> ri_to_c/2
  FFT/3 -> Delay2/1, spect_cnt2/1, spect_cnt1/2, acc_cntrl/2(sync)
  ri_to_c/1 -> power_calc/1(pol0)
  FFT1/2 -> Convert4/1
  [adc_dq] -> FFT1/1
  spect_cnt4/1 -> fft_sync_inc1/1(out_reg)
  ri_to_c1/1 -> power_calc/2(pol1)
  FFT1/3 -> Delay3/1
  Convert4/1 -> ri_to_c1/2
  Constant12/1 -> FFT1/2
  [sync_fft] -> FFT1/3
  FFT1/1 -> Convert3/1
  Convert3/1 -> ri_to_c1/1
  fft_sync_inc1/1(sim_out_reg) -> Terminator10/1
  fft_sync_inc0/1(sim_out_reg) -> Terminator9/1
  Delay3/1 -> spect_cnt4/1
  adc_voltage_snap/1(arm_out) -> Terminator5/1
  Delay2/1 -> spect_cnt3/1
  [adc_dv] -> frame_cntr/2
  frame_cntr/1 -> Relational1/1
  Constant1/1 -> Relational1/2
  Relational1/1 -> [sync_fft]
  [rst] -> frame_cntr/1

== system rp_spectrometer/acc_cnt ==
  out_reg : Inport
  assert_reg : xbsIndex_r4/Assert  assert_type=on  type_source=Explicitly  gui_display_data_type=Fixed-point  arith_type=Unsigned  n_bits=32  bin_pt=0  preci_type=Single  exp_width=8  frac_width=24  assert_rate=off  rate_source=Explicitly  period=1  output_port=on  block_type=assert
  cast_gw : xbsIndex_r4/Convert  gui_display_data_type=Fixed-point  arith_type=Unsigned  n_bits=32  bin_pt=0  float_type=Single  exp_bits=8  fraction_bits=24  quantization=Truncate  overflow=Wrap  en=off  latency=1  pipeline=off  dbl_ovrd=off  block_type=convert
  io_delay : xbsIndex_r4/Delay  rst=off  infoeditControl=Selection of Reset will increase slice count due to use of real FFs and instead of SRLs  en=off  latency=0  reg_retiming=on  dbl_ovrd=off  block_type=delay
  reint1 : xbsIndex_r4/Reinterpret  force_arith_type=on  arith_type=Unsigned  force_bin_pt=on  bin_pt=0  block_type=reinterpret
  sim_out : Terminator
  sim_out_reg_gw : xbsIndex_r4/Gateway Out  inherit_from_input=off  hdl_port=off  rows=1  columns=1  UseAsDAC=off  DACChannel='1'  interface=None  automatic_assignment=on  address_offset=hex2dec('00')  intf_name=''  intf_description=''  timing_constraint=None  locs_specified=off  LOCs={}  io_standard={}  block_type=gatewayout
  sim_out_reg_sim_delay : xbsIndex_r4/Delay  rst=off  infoeditControl=Selection of Reset will increase slice count due to use of real FFs and instead of SRLs  en=off  latency=1  reg_retiming=on  dbl_ovrd=off  block_type=delay
  tut_spec_acc_cnt_user_data_in : xbsIndex_r4/Gateway Out  inherit_from_input=off  hdl_port=on  rows=1  columns=1  UseAsDAC=off  DACChannel='1'  interface=None  automatic_assignment=on  address_offset=hex2dec('00')  intf_name=''  intf_description=''  timing_constraint=None  locs_specified=off  LOCs={}  io_standard={}  block_type=gatewayout
  sim_out_reg : Outport  VectorParamsAs1DForOutWhenUnconnected=off
  wires:
  sim_out_reg_sim_delay/1 -> sim_out_reg_gw/1
  sim_out_reg_gw/1 -> sim_out_reg/1
  io_delay/1 -> cast_gw/1
  cast_gw/1 -> tut_spec_acc_cnt_user_data_in/1
  tut_spec_acc_cnt_user_data_in/1 -> sim_out/1
  out_reg/1 -> sim_out_reg_sim_delay/1, assert_reg/1
  assert_reg/1 -> reint1/1
  reint1/1 -> io_delay/1

== system rp_spectrometer/acc_cntrl ==
  acc_len : Inport
  sync : Inport  Port=2
  rst : Inport  Port=3
  Logical : xbsIndex_r4/Logical  logical_function=OR  inputs=2  en=off  latency=0  precision=Full  arith_type=Unsigned  n_bits=8  bin_pt=2  align_bp=on  dbl_ovrd=off  block_type=logical
      settings: xl_area=[0, 0, 0, 0, 0, 0, 0]
  Register : xbsIndex_r4/Register  init=0  rst=on  en=on  dbl_ovrd=off  block_type=register
      settings: xl_area=[0, 0, 0, 0, 0, 0, 0]
  Relational5 : xbsIndex_r4/Relational  mode=a=b  op_type=Bool  en=off  latency=0  dbl_ovrd=off  block_type=relational
      settings: xl_area=[0, 0, 0, 0, 0, 0, 0]  block_version=10.1.3
  Shift : xbsIndex_r4/Shift  shift_dir=Left  shift_bits=chan_bits  en=off  latency=0  precision=Full  arith_type="Signed  (2's comp)"  n_bits=8  bin_pt=2  quantization=Truncate  overflow=Wrap  dbl_ovrd=off  block_type=shift
      settings: xl_area=[0, 0, 0, 0, 0, 0, 0]  block_version=10.1.3
  cntr : xbsIndex_r4/Counter  cnt_type=Free Running  cnt_to=Inf  operation=Up  start_count=1  cnt_by_val=1  arith_type=Unsigned  n_bits=32  bin_pt=0  load_pin=off  rst=on  en=off  explicit_period=on  period=1  use_behavioral_HDL=on  implementation=Fabric  use_rpm=on  dbl_ovrd=off  block_type=counter
      settings: xl_area=[0, 0, 0, 0, 0, 0, 0]
  edge_detect : Subsystem  AncestorBlock=casper_library_misc/edge_detect  mask(edge_detect){edge=Rising, polarity=Active High, x_in=[0 0.08 0.08 0.16 0.16 0.24 0.24 0.32 0.32 0.4], y_in=[-1 -1  1  1  1  1  1  1  1  1], x_out=[0.6 0.68 0.68 0.76 0.76 0.84 0.84 0.92 0.92 1], y_out=[-1 -1  1  1 -1 -1 -1 -1 -1 -1]}
      mask prompts: edge "Edge Type"; polarity "Output Polarity"; x_in "Input X Positions"; y_in "Input Y Positions"; x_out "Output X Positions"; y_out "Output Y Positions"
      mask help: Output is active for one-cycle after each edge of the specified type (i.e. rising, falling or both).
      mask init: same as rp_spectrometer/edge_detect
      settings: AttributesFormatString=|
      | rising edges
      | active high
      mask Help: Output is active for one-cycle after each edge of the specified type (i.e. rising, falling, or both).  Latency is zero.
      mask TypeOptions edge: Rising | Falling | Both
      mask TypeOptions polarity: Active High | Active Low
      mask Display:
      | plot(x_in_num,0.5+y_in_num*0.2);
      | plot(x_out_num,0.5+y_out_num*0.2);
  pipeline15 : Subsystem  AncestorBlock=casper_library_delays/pipeline  mask(pipeline){csp_latency=1}
      mask prompts: csp_latency "Latency"
      mask help:
      | An explicitly laid-out delay line to avoid mapping to SRL16s
      | for use in pipelining to help achieve timing closure.
      mask init:
      | pipeline_init(gcb,'latency',csp_latency);
      settings: AttributesFormatString=Latency = %<latency>
      mask Display:
      | port_label('input', 1, 'd');
      | port_label('output', 1, 'q');
      | disp(['Z^-', num2str(csp_latency)]);
  new_acc : Outport  VectorParamsAs1DForOutWhenUnconnected=off
  wires:
  cntr/1 -> Relational5/1
  pipeline15/1(q) -> Relational5/2
  edge_detect/1(out) -> Logical/1
  Register/1 -> edge_detect/1(in)
  Logical/1 -> cntr/1
  acc_len/1 -> Shift/1
  Relational5/1 -> Logical/2, new_acc/1
  sync/1 -> Register/1, Register/3
  rst/1 -> Register/2
  Shift/1 -> pipeline15/1(d)
